simulink model "au50_hbm_data_test"  (R2021a)
settings: Solver=VariableStepDiscrete  StartTime=0.0  StopTime=3000  RelTol=1e-3
libraries: xbsIndex_r4 x618, casper_library_misc x3, xps_library x2
(part 5 of 10)

== system au50_hbm_data_test/hbm_in_rd_snap/ss/ctrl ==
  au50_hbm_data_test_hbm_in_rd_snap_ss_ctrl_user_data_out : xbsIndex_r4/Gateway In  gui_display_data_type=Fixed-point  arith_type=Unsigned  n_bits=32  bin_pt=0  preci_type=Single  exp_width=8  frac_width=24  rows=1  columns=1  quantization="Round  (unbiased: +/- Inf)"  overflow=Saturate  period=1  UseAsADC=off  ADCChannel='1'  interface=None  automatic_assignment=on  address_offset=hex2dec('00')  intf_name=''  intf_description=''  default_value=0  timing_constraint=None  locs_specified=off  LOCs={}  io_standard={}  inherit_from_input=off  hdl_port=on  dbl_ovrd=off  block_type=gatewayin
  convert1_1 : DataTypeConversion  OutDataTypeStr=fixdt('ufix32_En0')  LockScale=on
  convert2_1 : DataTypeConversion  OutDataTypeStr=fixdt('ufix32_En0')  ConvertRealWorld=Stored Integer (SI)  LockScale=on
  gain_1 : Gain  OutDataTypeStr=fixdt('ufix32_En0')
  io_delay : xbsIndex_r4/Delay  rst=off  infoeditControl=Selection of Reset will increase slice count due to use of real FFs and instead of SRLs  en=off  latency=0  reg_retiming=on  dbl_ovrd=off  block_type=delay
  reint1 : xbsIndex_r4/Reinterpret  force_arith_type=on  arith_type=Unsigned  force_bin_pt=on  bin_pt=0  block_type=reinterpret
  sim_1 : Constant  Value=0
  slice_reg : xbsIndex_r4/Slice  nbits=32  boolean_output=off  mode=Lower Bit Location + Width  bit1=0  base1=MSB of Input  bit0=0  base0=LSB of Input  dbl_ovrd=off  block_type=slice
  in_reg : Outport  VectorParamsAs1DForOutWhenUnconnected=off
  wires:
  au50_hbm_data_test_hbm_in_rd_snap_ss_ctrl_user_data_out/1 -> io_delay/1
  sim_1/1 -> convert1_1/1
  convert1_1/1 -> convert2_1/1
  convert2_1/1 -> gain_1/1
  gain_1/1 -> au50_hbm_data_test_hbm_in_rd_snap_ss_ctrl_user_data_out/1
  io_delay/1 -> slice_reg/1
  slice_reg/1 -> reint1/1
  reint1/1 -> in_reg/1

== system au50_hbm_data_test/hbm_in_rd_snap/ss/ctrl_combine ==
  in1 : Inport
  in2 : Inport  Port=2
  in3 : Inport  Port=3
  in4 : Inport  Port=4
  concatenate : xbsIndex_r4/Concat  num_inputs=4  dbl_ovrd=off  block_type=concat
  reinterpret{1..4} (4 alike) : xbsIndex_r4/Reinterpret  force_arith_type=on  arith_type=Unsigned  force_bin_pt=on  bin_pt=0  block_type=reinterpret
      reinterpret1 settings: infoedit="Changes signal type without altering the binary representation.   You can changed the signal between signed and unsigned, and relocate the binary point.<br><br>Hardware notes: In hardware this block costs nothing.<br><br>Example:  Suppose the input is 6 bits wide, signed, with 2 fractional bits, and the output is forced to unsigned with 0 fractional bits.  Then an input of -2.0 (1110.00 in binary 2's complement) becomes an output of 56 (111000 in binary)."
      reinterpret2 settings: infoedit="Changes signal type without altering the binary representation.   You can changed the signal between signed and unsigned, and relocate the binary point.<br><br>Hardware notes: In hardware this block costs nothing.<br><br>Example:  Suppose the input is 6 bits wide, signed, with 2 fractional bits, and the output is forced to unsigned with 0 fractional bits.  Then an input of -2.0 (1110.00 in binary 2's complement) becomes an output of 56 (111000 in binary)."
  bus_out : Outport  VectorParamsAs1DForOutWhenUnconnected=off
  wires:
  reinterpret4/1 -> concatenate/4
  in4/1 -> reinterpret4/1
  reinterpret3/1 -> concatenate/3
  in3/1 -> reinterpret3/1
  reinterpret2/1 -> concatenate/2
  in2/1 -> reinterpret2/1
  reinterpret1/1 -> concatenate/1
  in1/1 -> reinterpret1/1
  concatenate/1 -> bus_out/1

== system au50_hbm_data_test/hbm_in_rd_snap/ss/ctrl_split ==
  bus_in : Inport
  reinterpret2 : xbsIndex_r4/Reinterpret  force_arith_type=on  arith_type=Unsigned  force_bin_pt=on  bin_pt=0  block_type=reinterpret
  reinterpret4 : xbsIndex_r4/Reinterpret  force_arith_type=on  arith_type=Unsigned  force_bin_pt=on  bin_pt=0  block_type=reinterpret
  slice1 : xbsIndex_r4/Slice  nbits=1  boolean_output=on  mode=Upper Bit Location + Width  bit1=-31  base1=MSB of Input  bit0=0  base0=LSB of Input  dbl_ovrd=off  block_type=slice
  slice2 : xbsIndex_r4/Slice  nbits=2  boolean_output=off  mode=Upper Bit Location + Width  bit1=-29  base1=MSB of Input  bit0=0  base0=LSB of Input  dbl_ovrd=off  block_type=slice
  slice3 : xbsIndex_r4/Slice  nbits=1  boolean_output=on  mode=Upper Bit Location + Width  bit1=-28  base1=MSB of Input  bit0=0  base0=LSB of Input  dbl_ovrd=off  block_type=slice
  slice4 : xbsIndex_r4/Slice  nbits=28  boolean_output=off  mode=Upper Bit Location + Width  bit1=0  base1=MSB of Input  bit0=0  base0=LSB of Input  dbl_ovrd=off  block_type=slice
  msb_out4 : Outport  VectorParamsAs1DForOutWhenUnconnected=off
  out3 : Outport  Port=2  VectorParamsAs1DForOutWhenUnconnected=off
  out2 : Outport  Port=3  VectorParamsAs1DForOutWhenUnconnected=off
  lsb_out1 : Outport  Port=4  VectorParamsAs1DForOutWhenUnconnected=off
  wires:
  slice1/1 -> lsb_out1/1
  reinterpret2/1 -> out2/1
  slice2/1 -> reinterpret2/1
  slice3/1 -> out3/1
  reinterpret4/1 -> msb_out4/1
  slice4/1 -> reinterpret4/1
  bus_in/1 -> slice1/1, slice2/1, slice3/1, slice4/1

== system au50_hbm_data_test/hbm_in_rd_snap/ss/status ==
  out_reg : Inport
  assert_reg : xbsIndex_r4/Assert  assert_type=on  type_source=Explicitly  gui_display_data_type=Fixed-point  arith_type=Unsigned  n_bits=32  bin_pt=0  preci_type=Single  exp_width=8  frac_width=24  assert_rate=off  rate_source=Explicitly  period=1  output_port=on  block_type=assert
  au50_hbm_data_test_hbm_in_rd_snap_ss_status_user_data_in : xbsIndex_r4/Gateway Out  inherit_from_input=off  hdl_port=on  rows=1  columns=1  UseAsDAC=off  DACChannel='1'  interface=None  automatic_assignment=on  address_offset=hex2dec('00')  intf_name=''  intf_description=''  timing_constraint=None  locs_specified=off  LOCs={}  io_standard={}  block_type=gatewayout
  cast_gw : xbsIndex_r4/Convert  gui_display_data_type=Fixed-point  arith_type=Unsigned  n_bits=32  bin_pt=0  float_type=Single  exp_bits=8  fraction_bits=24  quantization=Truncate  overflow=Wrap  en=off  latency=1  pipeline=off  dbl_ovrd=off  block_type=convert
  io_delay : xbsIndex_r4/Delay  rst=off  infoeditControl=Selection of Reset will increase slice count due to use of real FFs and instead of SRLs  en=off  latency=0  reg_retiming=on  dbl_ovrd=off  block_type=delay
  reint1 : xbsIndex_r4/Reinterpret  force_arith_type=on  arith_type=Unsigned  force_bin_pt=on  bin_pt=0  block_type=reinterpret
  sim_out : Terminator
  wires:
  io_delay/1 -> cast_gw/1
  cast_gw/1 -> au50_hbm_data_test_hbm_in_rd_snap_ss_status_user_data_in/1
  au50_hbm_data_test_hbm_in_rd_snap_ss_status_user_data_in/1 -> sim_out/1
  out_reg/1 -> assert_reg/1
  assert_reg/1 -> reint1/1
  reint1/1 -> io_delay/1

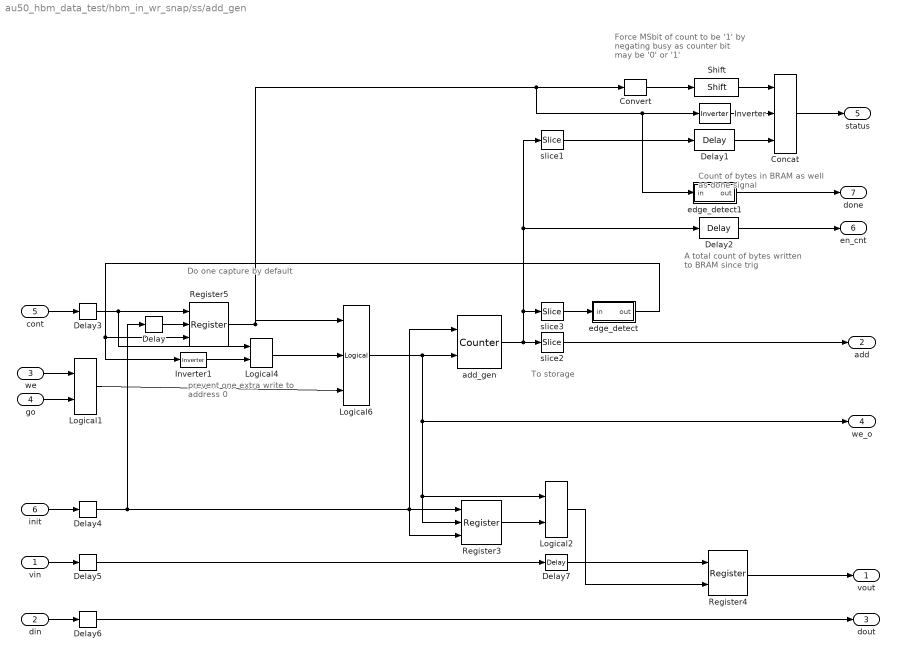
== system au50_hbm_data_test/hbm_in_wr_snap/ss/add_gen ==
  note: Force MSbit of count
      | to be '1' by negating busy
      | as counter bit may be '0' or '1'
  note: A total count of
      | bytes written to
      | BRAM since trig
  note: Count of bytes in BRAM
      | as well as done signal
  note: Do one
      | capture by
      | default
  note: prevent one extra
      | write to address 0
  note: To storage
  vin : Inport
  din : Inport  Port=2
  we : Inport  Port=3
  go : Inport  Port=4
  cont : Inport  Port=5
  init : Inport  Port=6
  Concat : xbsIndex_r4/Concat  num_inputs=3  dbl_ovrd=off  block_type=concat
      settings: block_version=10.1.3
  Convert : xbsIndex_r4/Convert  gui_display_data_type=Fixed-point  arith_type=Unsigned  n_bits=32-nsamples-log2(increment)-1  bin_pt=0  float_type=Single  exp_bits=8  fraction_bits=24  quantization=Truncate  overflow=Wrap  en=off  latency=0  pipeline=off  dbl_ovrd=off  block_type=convert
      settings: block_version=10.1.3
  Delay{,3..6} (5 alike) : xbsIndex_r4/Delay  rst=off  infoeditControl=Selection of Reset will increase slice count due to use of real FFs and instead of SRLs  en=off  latency=1  reg_retiming=on  dbl_ovrd=off  block_type=delay
      settings: block_version=11.4
  Delay1 : xbsIndex_r4/Delay  rst=off  infoeditControl=Selection of Reset will increase slice count due to use of real FFs and instead of SRLs  en=off  latency=1  reg_retiming=off  dbl_ovrd=off  block_type=delay
      settings: block_version=11.4
  Delay2 : xbsIndex_r4/Delay  rst=off  infoeditControl=Selection of Reset will increase slice count due to use of real FFs and instead of SRLs  en=off  latency=1  reg_retiming=off  dbl_ovrd=off  block_type=delay
      settings: block_version=11.4
  Delay7 : xbsIndex_r4/Delay  rst=off  infoeditControl=Selection of Reset will increase slice count due to use of real FFs and instead of SRLs  en=off  latency=1  reg_retiming=off  dbl_ovrd=off  block_type=delay
      settings: block_version=11.4
  Inverter : xbsIndex_r4/Inverter  en=off  latency=1  dbl_ovrd=off  block_type=inv
      settings: block_version=11.4
  Inverter1 : xbsIndex_r4/Inverter  en=off  latency=0  dbl_ovrd=off  block_type=inv
      settings: block_version=11.4
  Logical1 : xbsIndex_r4/Logical  logical_function=AND  inputs=2  en=off  latency=1  precision=Full  arith_type=Unsigned  n_bits=8  bin_pt=2  align_bp=on  dbl_ovrd=off  block_type=logical
      settings: xl_area=[0, 0, 0, 0, 0, 0, 0]
  Logical2 : xbsIndex_r4/Logical  logical_function=AND  inputs=2  en=off  latency=1  precision=Full  arith_type=Unsigned  n_bits=8  bin_pt=2  align_bp=on  dbl_ovrd=off  block_type=logical
      settings: xl_area=[0, 0, 0, 0, 0, 0, 0]
  Logical4 : xbsIndex_r4/Logical  logical_function=OR  inputs=2  en=off  latency=0  precision=Full  arith_type=Unsigned  n_bits=8  bin_pt=2  align_bp=on  dbl_ovrd=off  block_type=logical
      settings: xl_area=[0, 0, 0, 0, 0, 0, 0]
  Logical6 : xbsIndex_r4/Logical  logical_function=AND  inputs=3  en=off  latency=0  precision=Full  arith_type=Unsigned  n_bits=8  bin_pt=2  align_bp=on  dbl_ovrd=off  block_type=logical
      settings: xl_area=[0, 0, 0, 0, 0, 0, 0]
  Register3 : xbsIndex_r4/Register  init=0  rst=on  en=on  dbl_ovrd=off  block_type=register
      settings: xl_area=[0, 0, 0, 0, 0, 0, 0]
  Register4 : xbsIndex_r4/Register  init=0  rst=off  en=on  dbl_ovrd=off  block_type=register
      settings: xl_area=[0, 0, 0, 0, 0, 0, 0]
  Register5 : xbsIndex_r4/Register  init=1  rst=on  en=on  dbl_ovrd=off  block_type=register
      settings: xl_area=[0, 0, 0, 0, 0, 0, 0]
  Shift : xbsIndex_r4/Shift  shift_dir=Left  shift_bits=32-nsamples-log2(increment)-1-1  en=off  latency=1  precision=Full  arith_type="Signed  (2's comp)"  n_bits=16  bin_pt=14  quantization=Truncate  overflow=Wrap  dbl_ovrd=off  block_type=shift
  add_gen : xbsIndex_r4/Counter  cnt_type=Free Running  cnt_to=1  operation=Up  start_count=0  cnt_by_val=increment  arith_type=Unsigned  n_bits=counter_size  bin_pt=0  load_pin=off  rst=on  en=on  explicit_period=on  period=1  use_behavioral_HDL=off  implementation=DSP48  use_rpm=on  dbl_ovrd=off  block_type=counter
      settings: xl_area=[0, 0, 0, 0, 0, 0, 0]
  edge_detect : Subsystem  AncestorBlock=casper_library_misc/edge_detect  mask(edge_detect){edge=Both, polarity=Active High, x_in=[0 0.08 0.08 0.16 0.16 0.24 0.24 0.32 0.32 0.4], y_in=[-1 -1  1  1  1  1 -1 -1 -1 -1], x_out=[0.6 0.68 0.68 0.76 0.76 0.84 0.84 0.92 0.92 1], y_out=[-1 -1  1  1 -1 -1  1  1 -1 -1]}
      mask prompts: edge "Edge Type"; polarity "Output Polarity"; x_in "Input X Positions"; y_in "Input Y Positions"; x_out "Output X Positions"; y_out "Output Y Positions"
      mask help: Output is active for one-cycle after each edge of the specified type (i.e. rising, falling or both).
      mask init: same as au50_hbm_data_test/edge_detect1
      settings: AttributesFormatString=|
      | both edges
      | active high
      mask Help: Output is active for one-cycle after each edge of the specified type (i.e. rising, falling, or both).  Latency is zero.
      mask TypeOptions edge: Rising | Falling | Both
      mask TypeOptions polarity: Active High | Active Low
      mask Display:
      | plot(x_in_num,0.5+y_in_num*0.2);
      | plot(x_out_num,0.5+y_out_num*0.2);
  edge_detect1 : Subsystem  AncestorBlock=casper_library_scopes/snapshot/add_gen/edge_detect  mask(edge_detect){edge=Both, polarity=Active High, x_in=[0 0.08 0.08 0.16 0.16 0.24 0.24 0.32 0.32 0.4], y_in=[-1 -1  1  1  1  1 -1 -1 -1 -1], x_out=[0.6 0.68 0.68 0.76 0.76 0.84 0.84 0.92 0.92 1], y_out=[-1 -1  1  1 -1 -1  1  1 -1 -1]}
      mask prompts: edge "Edge Type"; polarity "Output Polarity"; x_in "Input X Positions"; y_in "Input Y Positions"; x_out "Output X Positions"; y_out "Output Y Positions"
      mask help: Output is active for one-cycle after each edge of the specified type (i.e. rising, falling or both).
      mask init: same as au50_hbm_data_test/edge_detect1
      settings: AttributesFormatString=|
      | both edges
      | active high
      mask Help: Output is active for one-cycle after each edge of the specified type (i.e. rising, falling, or both).  Latency is zero.
      mask TypeOptions edge: Rising | Falling | Both
      mask TypeOptions polarity: Active High | Active Low
      mask Display:
      | plot(x_in_num,0.5+y_in_num*0.2);
      | plot(x_out_num,0.5+y_out_num*0.2);
  slice1 : xbsIndex_r4/Slice  nbits=nsamples+log2(increment)  boolean_output=off  mode=Lower Bit Location + Width  bit1=0  base1=LSB of Input  bit0=0  base0=LSB of Input  dbl_ovrd=off  block_type=slice
      settings: block_version=10.1.3
  slice2 : xbsIndex_r4/Slice  nbits=nsamples-burst_size  boolean_output=off  mode=Lower Bit Location + Width  bit1=0  base1=LSB of Input  bit0=log2(increment)+burst_size  base0=LSB of Input  dbl_ovrd=off  block_type=slice
      settings: block_version=10.1.3
  slice3 : xbsIndex_r4/Slice  nbits=1  boolean_output=on  mode=Lower Bit Location + Width  bit1=0  base1=MSB of Input  bit0=nsamples + log2(increment)  base0=LSB of Input  dbl_ovrd=off  block_type=slice
      settings: block_version=10.1.3
  vout : Outport  VectorParamsAs1DForOutWhenUnconnected=off
  add : Outport  Port=2  VectorParamsAs1DForOutWhenUnconnected=off
  dout : Outport  Port=3  VectorParamsAs1DForOutWhenUnconnected=off
  we_o : Outport  Port=4  VectorParamsAs1DForOutWhenUnconnected=off
  status : Outport  Port=5  VectorParamsAs1DForOutWhenUnconnected=off
  en_cnt : Outport  Port=6  VectorParamsAs1DForOutWhenUnconnected=off
  done : Outport  Port=7  VectorParamsAs1DForOutWhenUnconnected=off
  wires:
  Delay6/1 -> dout/1
  Delay5/1 -> Delay7/1
  Delay4/1 -> Delay/1, Register3/1, Register3/3, add_gen/1
  Delay3/1 -> Register5/1, Logical4/1
  Delay7/1 -> Register4/1
  Logical1/1 -> Logical6/3
  go/1 -> Logical1/2
  we/1 -> Logical1/1
  Logical4/1 -> Logical6/2
  Inverter/1 -> Concat/2
  slice1/1 -> Delay1/1
  Delay1/1 -> Concat/3
  din/1 -> Delay6/1
  Delay2/1 -> en_cnt/1
  slice2/1 -> add/1
  Convert/1 -> Shift/1
  Concat/1 -> status/1
  Logical6/1 -> add_gen/2, Register3/2, Logical2/1, we_o/1
  init/1 -> Delay4/1
  slice3/1 -> edge_detect/1(in)
  Register5/1 -> Logical6/1, edge_detect1/1(in), Inverter/1, Convert/1
  add_gen/1 -> slice3/1, Delay2/1, slice1/1, slice2/1
  vin/1 -> Delay5/1
  Register3/1 -> Logical2/2
  Logical2/1 -> Register4/2
  Register4/1 -> vout/1
  edge_detect/1(out) -> Register5/3, Inverter1/1
  cont/1 -> Delay3/1
  Inverter1/1 -> Logical4/2
  Delay/1 -> Register5/2
  Shift/1 -> Concat/1
  edge_detect1/1(out) -> done/1

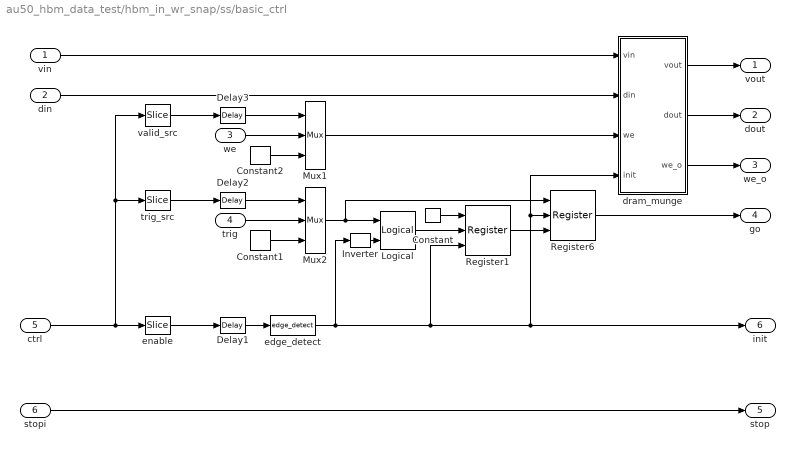
== system au50_hbm_data_test/hbm_in_wr_snap/ss/basic_ctrl ==
  vin : Inport
  din : Inport  Port=2
  we : Inport  Port=3
  trig : Inport  Port=4
  ctrl : Inport  Port=5
  stopi : Inport  Port=6
  Constant : xbsIndex_r4/Constant  const=1  gui_display_data_type=Fixed-point  arith_type=Boolean  n_bits=16  bin_pt=14  preci_type=Single  exp_width=8  frac_width=24  explicit_period=on  period=1  equ=P=C  opselect=C  inp2=PCIN>>17  opr=+  inp1=P  carry=CIN  dbl_ovrd=off  block_type=constant
      settings: block_version=11.4
  Constant1 : xbsIndex_r4/Constant  const=1  gui_display_data_type=Fixed-point  arith_type=Boolean  n_bits=1  bin_pt=0  preci_type=Single  exp_width=8  frac_width=24  explicit_period=on  period=1  equ=P=C  opselect=C  inp2=PCIN>>17  opr=+  inp1=P  carry=CIN  dbl_ovrd=off  block_type=constant
  Constant2 : xbsIndex_r4/Constant  const=1  gui_display_data_type=Fixed-point  arith_type=Boolean  n_bits=1  bin_pt=0  preci_type=Single  exp_width=8  frac_width=24  explicit_period=on  period=1  equ=P=C  opselect=C  inp2=PCIN>>17  opr=+  inp1=P  carry=CIN  dbl_ovrd=off  block_type=constant
  Delay1 : xbsIndex_r4/Delay  rst=off  infoeditControl=Selection of Reset will increase slice count due to use of real FFs and instead of SRLs  en=off  latency=1  reg_retiming=off  dbl_ovrd=off  block_type=delay
      settings: block_version=11.4
  Delay2 : xbsIndex_r4/Delay  rst=off  infoeditControl=Selection of Reset will increase slice count due to use of real FFs and instead of SRLs  en=off  latency=1  reg_retiming=off  dbl_ovrd=off  block_type=delay
      settings: block_version=11.4
  Delay3 : xbsIndex_r4/Delay  rst=off  infoeditControl=Selection of Reset will increase slice count due to use of real FFs and instead of SRLs  en=off  latency=1  reg_retiming=off  dbl_ovrd=off  block_type=delay
      settings: block_version=11.4
  Inverter : xbsIndex_r4/Inverter  en=off  latency=0  dbl_ovrd=off  block_type=inv
      settings: block_version=11.4
  Logical : xbsIndex_r4/Logical  logical_function=AND  inputs=2  en=off  latency=0  precision=Full  arith_type=Unsigned  n_bits=16  bin_pt=0  align_bp=on  dbl_ovrd=off  block_type=logical
      settings: block_version=11.4
  Mux1 : xbsIndex_r4/Mux  inputs=2  en=off  latency=0  precision=Full  arith_type="Signed  (2's comp)"  n_bits=8  bin_pt=2  quantization=Truncate  overflow=Wrap  dbl_ovrd=off  block_type=mux
      settings: xl_area=[0, 0, 0, 0, 0, 0, 0]
  Mux2 : xbsIndex_r4/Mux  inputs=2  en=off  latency=0  precision=Full  arith_type="Signed  (2's comp)"  n_bits=8  bin_pt=2  quantization=Truncate  overflow=Wrap  dbl_ovrd=off  block_type=mux
      settings: xl_area=[0, 0, 0, 0, 0, 0, 0]
  Register1 : xbsIndex_r4/Register  init=0  rst=on  en=on  dbl_ovrd=off  block_type=register
      settings: xl_area=[0, 0, 0, 0, 0, 0, 0]
  Register6 : xbsIndex_r4/Register  init=0  rst=on  en=on  dbl_ovrd=off  block_type=register
      settings: xl_area=[0, 0, 0, 0, 0, 0, 0]
  dram_munge : Subsystem  mask{dram=off, data_width=data_width}
      mask prompts: data_width "data width"
      mask init: same as au50_hbm_data_test/hbm_in_rd_snap/ss/basic_ctrl/dram_munge
  edge_detect : casper_library_misc/edge_detect  edge=Rising  polarity=Active High  x_in=[0 0.08 0.08 0.16 0.16 0.24 0.24 0.32 0.32 0.4]  y_in="[-1 -1  1  1  1  1  1  1  1  1]"  x_out=[0.6 0.68 0.68 0.76 0.76 0.84 0.84 0.92 0.92 1]  y_out="[-1 -1  1  1 -1 -1 -1 -1 -1 -1]"
  enable : xbsIndex_r4/Slice  nbits=1  boolean_output=on  mode=Lower Bit Location + Width  bit1=0  base1=LSB of Input  bit0=0  base0=LSB of Input  dbl_ovrd=off  block_type=slice
      settings: infoedit="Extracts a given range of bits from each input sample and presents it at the output.  The output type is ordinarily unsigned with binary point at zero, but can be Boolean when the slice is one bit wide.<P><P>Hardware notes: In hardware this block costs nothing."  block_version=10.1.3
  trig_src : xbsIndex_r4/Slice  nbits=1  boolean_output=on  mode=Lower Bit Location + Width  bit1=0  base1=LSB of Input  bit0=1  base0=LSB of Input  dbl_ovrd=off  block_type=slice
      settings: infoedit="Extracts a given range of bits from each input sample and presents it at the output.  The output type is ordinarily unsigned with binary point at zero, but can be Boolean when the slice is one bit wide.<P><P>Hardware notes: In hardware this block costs nothing."  block_version=10.1.3
  valid_src : xbsIndex_r4/Slice  nbits=1  boolean_output=on  mode=Lower Bit Location + Width  bit1=0  base1=LSB of Input  bit0=2  base0=LSB of Input  dbl_ovrd=off  block_type=slice
      settings: infoedit="Extracts a given range of bits from each input sample and presents it at the output.  The output type is ordinarily unsigned with binary point at zero, but can be Boolean when the slice is one bit wide.<P><P>Hardware notes: In hardware this block costs nothing."  block_version=10.1.3
  vout : Outport  VectorParamsAs1DForOutWhenUnconnected=off
  dout : Outport  Port=2  VectorParamsAs1DForOutWhenUnconnected=off
  we_o : Outport  Port=3  VectorParamsAs1DForOutWhenUnconnected=off
  go : Outport  Port=4  VectorParamsAs1DForOutWhenUnconnected=off
  stop : Outport  Port=5  VectorParamsAs1DForOutWhenUnconnected=off
  init : Outport  Port=6  VectorParamsAs1DForOutWhenUnconnected=off
  wires:
  Delay1/1 -> edge_detect/1
  Delay3/1 -> Mux1/1
  Delay2/1 -> Mux2/1
  dram_munge/1(vout) -> vout/1
  vin/1 -> dram_munge/1(vin)
  dram_munge/3(we_o) -> we_o/1
  dram_munge/2(dout) -> dout/1
  din/1 -> dram_munge/2(din)
  Inverter/1 -> Logical/2
  Mux2/1 -> Logical/1, Register6/1
  Register6/1 -> go/1
  trig/1 -> Mux2/2
  Mux1/1 -> dram_munge/3(we)
  we/1 -> Mux1/2
  ctrl/1 -> enable/1, valid_src/1, trig_src/1
  edge_detect/1 -> Inverter/1, Register1/3, dram_munge/4(init), Register6/2, init/1
  enable/1 -> Delay1/1
  Constant1/1 -> Mux2/3
  Constant2/1 -> Mux1/3
  trig_src/1 -> Delay2/1
  valid_src/1 -> Delay3/1
  Constant/1 -> Register1/1
  Register1/1 -> Register6/3
  Logical/1 -> Register1/2
  stopi/1 -> stop/1
